simulink model "prueba"  (R2025b)
settings: Solver=VariableStepAuto  StartTime=0.0  StopTime=10.0  RelTol=1e-3
values from neighbouring files (symbols this model uses):
  bcx = 1.0e6    (= 1000000)    [parametros.m]
  bcy = 10.0e6    (= 10000000)    [parametros.m]
  bh_eq = bhm + bhd/(ih^2)    (= 18.0165289256)    [parametros.m]
  bhb = 100e6    (= 100000000)    [parametros.m]
  bhEb = 2.2e9    (= 2200000000)    [parametros.m]
  bhwu = 150    [parametros.m]
  bt = 90.0    (= 90)    [parametros.m]
  bt_eq = btm + btd/(it^2)    (= 6.002)    [parametros.m]
  btb = 5.0e6    (= 5000000)    [parametros.m]
  btw = 3.0e3    (= 3000)    [parametros.m]
  g = 9.80665    [parametros.m]
  Hc = 2.59    [parametros.m]
  ih = 22.0    (= 22)    [parametros.m]
  it = 30.0    (= 30)    [parametros.m]
  Jh_eq = J_hm_hb + J_hd_hEb/(ih^2)    (= 37.8512396694)    [parametros.m]
  Jt_eq = Jtm_tb + Jtd/(it^2)    (= 8.33333333333)    [parametros.m]
  Kcy = 1.8e9    (= 1800000000)    [parametros.m]
  khwu = 236e6    (= 236000000)    [parametros.m]
  Ki_h = (wn_h^2)*Jh_eq    (= 34.1607438017)    [parametros.m]
  Ki_t = (wn_t^2*Mt)/Kf    (= 320)    [parametros.m]
  Kp_h = 2*zitta_h*wn_h*Jh_eq    (= 79.1090909091)    [parametros.m]
  Kp_t = (2*zitta_t*wn_t*Mt)/Kf    (= 1120)    [parametros.m]
  Ktw = 480e3    (= 480000)    [parametros.m]
  Lh0 = 110    [parametros.m]
  lh_0 = Yt0 - yh_0    (= 25)    [parametros.m]
  Mc_max = 50000    [parametros.m]
  Ms = 15000    [parametros.m]
  Mt = 30000    [parametros.m]
  rhd = 0.75    [parametros.m]
  rtd = 0.50    (= 0.5)    [parametros.m]
  tau_hm = 1.0e-3    (= 0.001)    [parametros.m]
  tau_tm = 1.0e-3    (= 0.001)    [parametros.m]
  Thb_Max = 50e3    (= 50000)    [parametros.m]
  ThEb_Max = 1.1e6    (= 1100000)    [parametros.m]
  Thm_0 = Ms*g*rhd/(2*ih)    (= 2507.38210227)    [parametros.m]
  Thm_Max = 20e3    (= 20000)    [parametros.m]
  titahm_0 = yh_0/(rhd/(2*ih))    (= 1173.33333333)    [parametros.m]
  titatm_0 = xtd_0/(rtd/it)    (= 1500)    [parametros.m]
  Ts2 = 1e-3    (= 0.001)    [parametros.m]
  Ttb_Max = 5.0e3    (= 5000)    [parametros.m]
  Ttm_0 = 0    [parametros.m]
  Ttm_Max = 4.0e3    (= 4000)    [parametros.m]
  vlx_0 = 0    [parametros.m]
  vly_0 = 0    [parametros.m]
  vt_0 = 0    [parametros.m]
  whm_0 = 0    [parametros.m]
  whm_rated = vh_nom*2*ih/rhd    (= 88)    [parametros.m]
  wtm_0 = 0    [parametros.m]
  xl_0 = xt_0    (= 25)    [parametros.m]
  xt_0 = 25    [parametros.m]
  xtd_0 = xt_0    (= 25)    [parametros.m]
  yl_0 = Yt0 - l_0    (= 19.975067839)    [parametros.m]
  Yt0 = 45.0    (= 45)    [parametros.m]
undefined symbols (not defined in the file or in its folder): DiscIntNeverNeededParam, magnitude
libraries: simulink x1
settings Model: Creator=lauta  LastModifiedBy=lauta

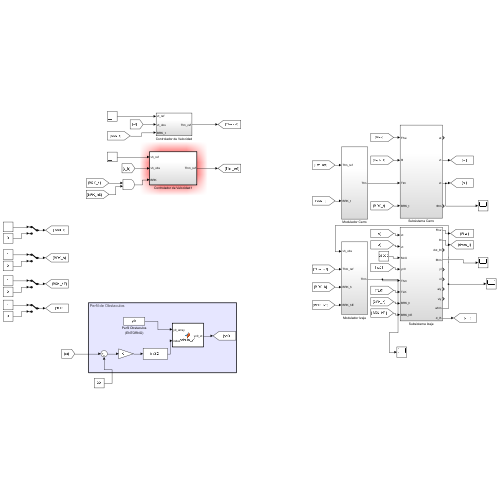
[thumbnail: Simulink's stored preview of the top-level diagram]
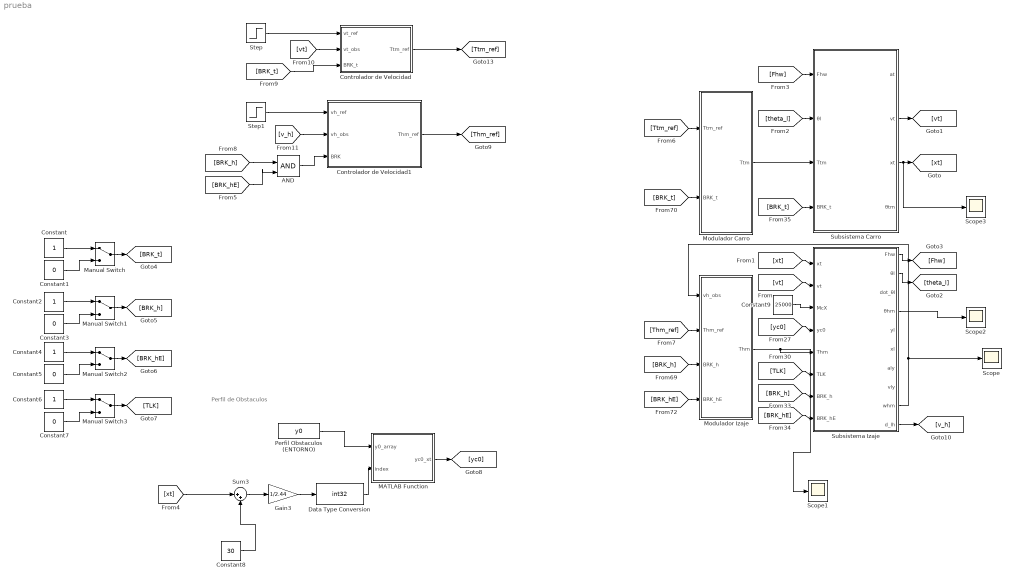
== system prueba ==
  note: Perfil de Obstaculos
  AND : Logic  IconShape=distinctive  AllPortsSameDT=off  OutDataTypeStr=boolean
  Constant{,2,4,6} (4 alike) : Constant
  Constant{1,3,5,7} (4 alike) : Constant  Value=0
  Constant8 : Constant  Value=30
  Constant9 : Constant  Value=25000
  Controlador de Velocidad : Subsystem
  Controlador de Velocidad1 : Subsystem  TreatAsAtomicUnit=on  SystemSampleTime=Ts2
  Data Type Conversion : DataTypeConversion  OutDataTypeStr=int32  RndMeth=Ceiling  SaturateOnIntegerOverflow=off
  Gain3 : Gain  Gain=1/2.44
  MATLAB Function : MATLAB Function  TreatAsAtomicUnit=on
  Manual Switch{,1..3} (4 alike) : ManualSwitch
  Modulador Carro : Subsystem
  Modulador Izaje : Subsystem
  Perfil Obstaculos (ENTORNO) : FromWorkspace  VariableName=y0
  Scope{,1..3} (4 alike) : Scope
      Scope settings: ActiveDisplayYMinimum=-16.360074628289411  ActiveDisplayYMaximum=147.24067165460474
      Scope1 settings: ActiveDisplayYMinimum=-1  ActiveDisplayYMaximum=1
      Scope2 settings: ActiveDisplayYMinimum=-1  ActiveDisplayYMaximum=1  DataLoggingVariableName=ScopeData2
      Scope3 settings: ActiveDisplayYMinimum=24.75610602663804  ActiveDisplayYMaximum=27.195045760257642  DataLoggingVariableName=ScopeData4
  Step : Step  SampleTime=0
  Step1 : Step  SampleTime=0
  Subsistema Carro : Subsystem
  Subsistema Izaje : Subsystem
  Sum3 : Sum  Inputs=|++
  wires:
  Subsistema Izaje/1(Fhw) -> [Fhw]
  Subsistema Izaje/9(whm) -> Scope/1, Modulador Izaje/1(vh_obs)
  [vt] -> Subsistema Izaje/2(vt)
  [BRK_t] -> Subsistema Carro/4(BRK_t)
  [xt] -> Subsistema Izaje/1(xt)
  Constant9/1 -> Subsistema Izaje/3(McX)
  Modulador Izaje/1(Thm) -> Scope1/1, Subsistema Izaje/5(Thm)
  [BRK_h] -> Subsistema Izaje/7(BRK_h)
  Subsistema Izaje/2(θl) -> [theta_l]
  Subsistema Carro/2(vt) -> [vt]
  [Fhw] -> Subsistema Carro/1(Fhw)
  [BRK_hE] -> Subsistema Izaje/8(BRK_hE)
  [theta_l] -> Subsistema Carro/2(θl)
  [BRK_h] -> Modulador Izaje/3(BRK_h)
  [yc0] -> Subsistema Izaje/4(yc0)
  [BRK_t] -> Modulador Carro/2(BRK_t)
  Subsistema Carro/3(xt) -> Scope3/1, [xt]
  [BRK_hE] -> Modulador Izaje/4(BRK_hE)
  Modulador Carro/1(Ttm) -> Subsistema Carro/3(Ttm)
  [TLK] -> Subsistema Izaje/6(TLK)
  Manual Switch/1 -> [BRK_t]
  Constant/1 -> Manual Switch/1
  Constant1/1 -> Manual Switch/2
  Constant3/1 -> Manual Switch1/2
  Constant2/1 -> Manual Switch1/1
  Manual Switch1/1 -> [BRK_h]
  Manual Switch2/1 -> [BRK_hE]
  Constant4/1 -> Manual Switch2/1
  Constant5/1 -> Manual Switch2/2
  Constant7/1 -> Manual Switch3/2
  Constant6/1 -> Manual Switch3/1
  Manual Switch3/1 -> [TLK]
  Gain3/1 -> Data Type Conversion/1
  Sum3/1 -> Gain3/1
  Perfil Obstaculos (ENTORNO)/1 -> MATLAB Function/1(y0_array)
  Data Type Conversion/1 -> MATLAB Function/2(index)
  [xt] -> Sum3/1
  Constant8/1 -> Sum3/2
  MATLAB Function/1(yc0_xt) -> [yc0]
  Subsistema Izaje/4(θhm) -> Scope2/1
  [Ttm_ref] -> Modulador Carro/1(Ttm_ref)
  [Thm_ref] -> Modulador Izaje/2(Thm_ref)
  Controlador de Velocidad/1(Ttm_ref) -> [Ttm_ref]
  Controlador de Velocidad1/1(Thm_ref) -> [Thm_ref]
  AND/1 -> Controlador de Velocidad1/3(BRK)
  [BRK_t] -> Controlador de Velocidad/3(BRK_t)
  [BRK_h] -> AND/1
  [BRK_hE] -> AND/2
  Step/1 -> Controlador de Velocidad/1(vt_ref)
  Step1/1 -> Controlador de Velocidad1/1(vh_ref)
  [vt] -> Controlador de Velocidad/2(vt_obs)
  Subsistema Izaje/10(d_lh) -> [v_h]
  [v_h] -> Controlador de Velocidad1/2(vh_obs)

== system prueba/Controlador de Velocidad ==
  vt_ref : Inport
  vt_obs : Inport  Port=2
  BRK_t : Inport  Port=3
  Discrete-Time Integrator : DiscreteIntegrator  IntegratorMethod=Integration: Trapezoidal  ExternalReset=level  SampleTime=-1  ICPrevOutput=DiscIntNeverNeededParam  ICPrevScaledInput=DiscIntNeverNeededParam
  Gain5 : Gain  Gain=Ki_t
  Gain6 : Gain  Gain=Kp_t
  NOT : Logic  Operator=NOT  IconShape=distinctive  AllPortsSameDT=off  OutDataTypeStr=boolean
  Sum6 : Sum  Inputs=+-
  Sum7 : Sum  Inputs=++|
  Ttm_ref : Outport
  wires:
  Sum6/1 -> Gain6/1, Discrete-Time Integrator/1  "e_v"
  Sum7/1 -> Ttm_ref/1
  Gain5/1 -> Sum7/2
  vt_ref/1 -> Sum6/1
  Gain6/1 -> Sum7/1
  vt_obs/1 -> Sum6/2
  Discrete-Time Integrator/1 -> Gain5/1
  BRK_t/1 -> NOT/1
  NOT/1 -> Discrete-Time Integrator/2

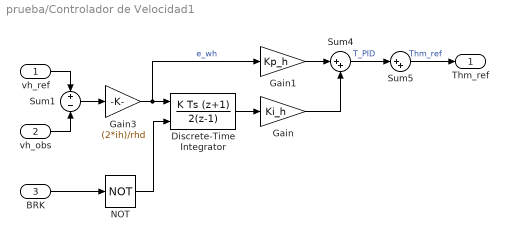
== system prueba/Controlador de Velocidad1 ==
  vh_ref : Inport
  vh_obs : Inport  Port=2
  BRK : Inport  Port=3
  Discrete-Time Integrator : DiscreteIntegrator  IntegratorMethod=Integration: Trapezoidal  ExternalReset=level  SampleTime=-1  ICPrevOutput=DiscIntNeverNeededParam  ICPrevScaledInput=DiscIntNeverNeededParam
  Gain : Gain  Gain=Ki_h
  Gain1 : Gain  Gain=Kp_h
  Gain3 : Gain  Gain=(2*ih)/rhd
  NOT : Logic  Operator=NOT  IconShape=distinctive  AllPortsSameDT=off  OutDataTypeStr=boolean
  Sum1 : Sum  Inputs=+-
  Sum4 : Sum  Inputs=|++
  Sum5 : Sum  Inputs=|++
  Thm_ref : Outport
  wires:
  Gain1/1 -> Sum4/1
  Sum1/1 -> Gain3/1
  vh_obs/1 -> Sum1/2
  Sum5/1 -> Thm_ref/1  "Thm_ref"
  Sum4/1 -> Sum5/1  "T_PID"
  vh_ref/1 -> Sum1/1
  Discrete-Time Integrator/1 -> Gain/1
  Gain/1 -> Sum4/2
  NOT/1 -> Discrete-Time Integrator/2
  BRK/1 -> NOT/1
  Gain3/1 -> Discrete-Time Integrator/1, Gain1/1  "e_wh"

== system prueba/Modulador Carro ==
  Ttm_ref : Inport
  BRK_t : Inport  Port=2
  Constant1 : Constant  Value=0
  Gain2 : Gain  Gain=1/tau_tm
  Integrator : Integrator  InitialCondition=Ttm_0
  Saturation : Saturate  UpperLimit=Ttm_Max  LowerLimit=-Ttm_Max
  Sum : Sum  Inputs=|+-
  Switch : Switch  Criteria=u2 > Threshold  SaturateOnIntegerOverflow=off  InputSameDT=off
  Ttm : Outport
  wires:
  Saturation/1 -> Sum/1  "Ttm_lim"
  Sum/1 -> Gain2/1
  Gain2/1 -> Integrator/1
  Integrator/1 -> Ttm/1, Sum/2
  Ttm_ref/1 -> Switch/1
  BRK_t/1 -> Switch/2
  Switch/1 -> Saturation/1
  Constant1/1 -> Switch/3

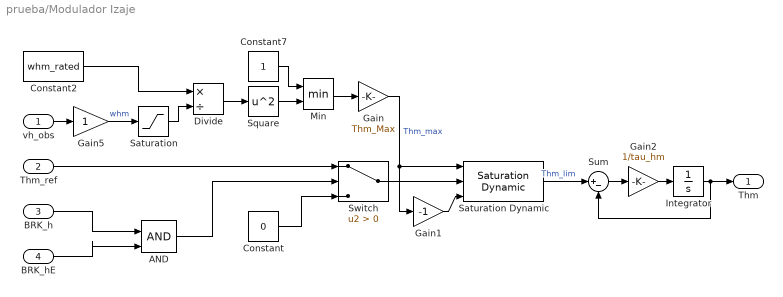
== system prueba/Modulador Izaje ==
  vh_obs : Inport
  Thm_ref : Inport  Port=2
  BRK_h : Inport  Port=3
  BRK_hE : Inport  Port=4
  AND : Logic  IconShape=distinctive  AllPortsSameDT=off  OutDataTypeStr=boolean
  Constant : Constant  Value=0
  Constant2 : Constant  Value=whm_rated
  Constant7 : Constant
  Divide : Product  Inputs=*/
  Gain : Gain  Gain=Thm_Max
  Gain1 : Gain  Gain=-1
  Gain2 : Gain  Gain=1/tau_hm
  Gain5 : Gain
  Integrator : Integrator  InitialCondition=Thm_0
  Min : MinMax  Inputs=2
  Saturation : Saturate  UpperLimit=inf  LowerLimit=whm_rated
  Saturation Dynamic : simulink/Discontinuities/Saturation Dynamic  OutMin=[]  OutMax=[]  OutDataTypeStr=Inherit: Same as second input  OutDataType=fixdt(1, 16)  OutScaling=2^-10  DoSatur=off
  Square : Math  Operator=square
  Sum : Sum  Inputs=|+-
  Switch : Switch  Criteria=u2 > Threshold  SaturateOnIntegerOverflow=off  InputSameDT=off
  Thm : Outport
  wires:
  Constant2/1 -> Divide/1
  Min/1 -> Gain/1
  Constant7/1 -> Min/1
  Gain/1 -> Gain1/1, Saturation Dynamic/1  "Thm_max"
  Saturation/1 -> Divide/2
  Square/1 -> Min/2
  Divide/1 -> Square/1
  vh_obs/1 -> Gain5/1
  Gain1/1 -> Saturation Dynamic/3
  Saturation Dynamic/1 -> Sum/1  "Thm_lim"
  Sum/1 -> Gain2/1
  Gain2/1 -> Integrator/1
  Integrator/1 -> Thm/1, Sum/2
  Thm_ref/1 -> Switch/1
  BRK_h/1 -> AND/1
  Switch/1 -> Saturation Dynamic/2
  BRK_hE/1 -> AND/2
  AND/1 -> Switch/2
  Gain5/1 -> Saturation/1  "whm"
  Constant/1 -> Switch/3

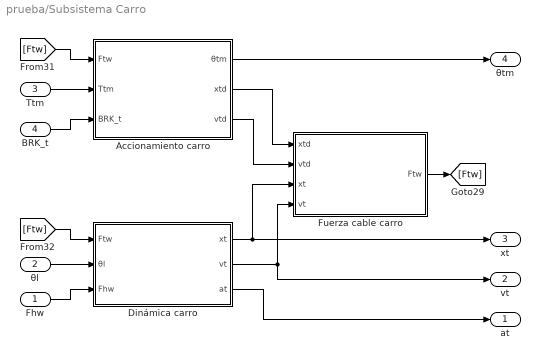
== system prueba/Subsistema Carro ==
  Fhw : Inport
  θl : Inport  Port=2
  Ttm : Inport  Port=3
  BRK_t : Inport  Port=4
  Accionamiento carro : Subsystem
  Dinámica carro : Subsystem
  Fuerza cable carro : Subsystem
  at : Outport
  vt : Outport  Port=2
  xt : Outport  Port=3
  θtm : Outport  Port=4
  wires:
  [Ftw] -> Accionamiento carro/1(Ftw)
  Accionamiento carro/1(θtm) -> θtm/1
  Dinámica carro/1(xt) -> Fuerza cable carro/3(xt), xt/1
  BRK_t/1 -> Accionamiento carro/3(BRK_t)
  [Ftw] -> Dinámica carro/1(Ftw)
  θl/1 -> Dinámica carro/2(θl)
  Ttm/1 -> Accionamiento carro/2(Ttm)
  Fuerza cable carro/1(Ftw) -> [Ftw]
  Dinámica carro/2(vt) -> Fuerza cable carro/4(vt), vt/1
  Accionamiento carro/2(xtd) -> Fuerza cable carro/1(xtd)
  Accionamiento carro/3(vtd) -> Fuerza cable carro/2(vtd)
  Fhw/1 -> Dinámica carro/3(Fhw)
  Dinámica carro/3(at) -> at/1

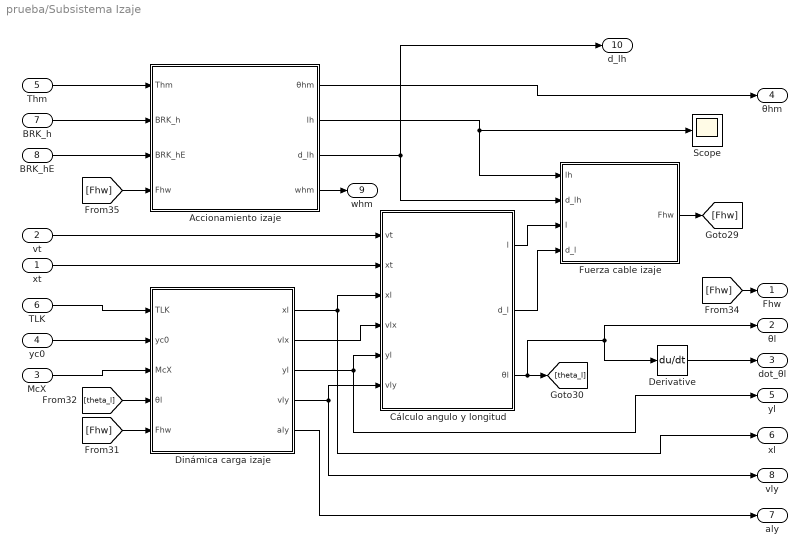
== system prueba/Subsistema Izaje ==
  xt : Inport
  vt : Inport  Port=2
  McX : Inport  Port=3
  yc0 : Inport  Port=4
  Thm : Inport  Port=5
  TLK : Inport  Port=6
  BRK_h : Inport  Port=7
  BRK_hE : Inport  Port=8
  Accionamiento izaje : Subsystem
  Cálculo angulo y longitud : Subsystem
  Derivative : Derivative
  Dinámica carga izaje : Subsystem
  Fuerza cable izaje : Subsystem
  Scope : Scope
      settings: ActiveDisplayYMinimum=-1  ActiveDisplayYMaximum=1  DataLoggingVariableName=ScopeData3
  Fhw : Outport
  θl : Outport  Port=2
  dot_θl : Outport  Port=3
  θhm : Outport  Port=4
  yl : Outport  Port=5
  xl : Outport  Port=6
  aly : Outport  Port=7
  vly : Outport  Port=8
  whm : Outport  Port=9
  d_lh : Outport  Port=10
  wires:
  vt/1 -> Cálculo angulo y longitud/1(vt)
  Accionamiento izaje/2(lh) -> Scope/1, Fuerza cable izaje/1(lh)
  yc0/1 -> Dinámica carga izaje/2(yc0)
  McX/1 -> Dinámica carga izaje/3(McX)
  Dinámica carga izaje/4(vly) -> vly/1, Cálculo angulo y longitud/6(vly)
  [Fhw] -> Accionamiento izaje/4(Fhw)
  [theta_l] -> Dinámica carga izaje/4(θl)
  xt/1 -> Cálculo angulo y longitud/2(xt)
  BRK_h/1 -> Accionamiento izaje/2(BRK_h)
  Dinámica carga izaje/1(xl) -> Cálculo angulo y longitud/3(xl), xl/1
  Dinámica carga izaje/2(vlx) -> Cálculo angulo y longitud/4(vlx)
  Fuerza cable izaje/1(Fhw) -> [Fhw]
  Cálculo angulo y longitud/1(l) -> Fuerza cable izaje/3(l)
  Accionamiento izaje/1(θhm) -> θhm/1
  Cálculo angulo y longitud/3(θl) -> θl/1, Derivative/1, [theta_l]
  TLK/1 -> Dinámica carga izaje/1(TLK)
  [Fhw] -> Dinámica carga izaje/5(Fhw)
  BRK_hE/1 -> Accionamiento izaje/3(BRK_hE)
  Thm/1 -> Accionamiento izaje/1(Thm)
  Dinámica carga izaje/3(yl) -> Cálculo angulo y longitud/5(yl), yl/1
  Cálculo angulo y longitud/2(d_l) -> Fuerza cable izaje/4(d_l)
  Accionamiento izaje/3(d_lh) -> d_lh/1, Fuerza cable izaje/2(d_lh)
  Dinámica carga izaje/5(aly) -> aly/1
  [Fhw] -> Fhw/1
  Derivative/1 -> dot_θl/1
  Accionamiento izaje/4(whm) -> whm/1

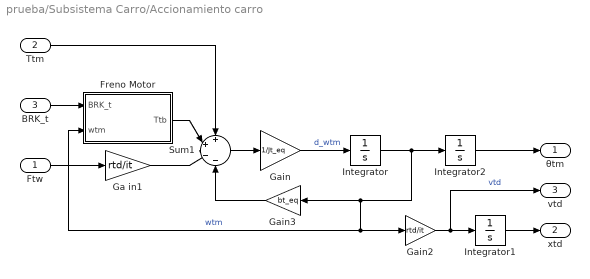
== system prueba/Subsistema Carro/Accionamiento carro ==
  Ftw : Inport
  Ttm : Inport  Port=2
  BRK_t : Inport  Port=3
  Freno Motor : Subsystem
  Ga in1 : Gain  Gain=rtd/it
  Gain : Gain  Gain=1/Jt_eq
  Gain2 : Gain  Gain=rtd/it
  Gain3 : Gain  Gain=bt_eq
  Integrator : Integrator  InitialCondition=wtm_0
  Integrator1 : Integrator  InitialCondition=xtd_0
  Integrator2 : Integrator  InitialCondition=titatm_0
  Sum1 : Sum  Inputs=++--
  θtm : Outport
  xtd : Outport  Port=2
  vtd : Outport  Port=3
  wires:
  Sum1/1 -> Gain/1
  Integrator/1 -> Gain2/1, Freno Motor/2(wtm), Gain3/1, Integrator2/1  "wtm"
  Gain2/1 -> Integrator1/1, vtd/1  "vtd"
  Ttm/1 -> Sum1/1
  Gain/1 -> Integrator/1  "d_wtm"
  BRK_t/1 -> Freno Motor/1(BRK_t)
  Integrator1/1 -> xtd/1
  Ftw/1 -> Ga in1/1
  Ga in1/1 -> Sum1/3
  Freno Motor/1(Ttb) -> Sum1/2
  Gain3/1 -> Sum1/4
  Integrator2/1 -> θtm/1

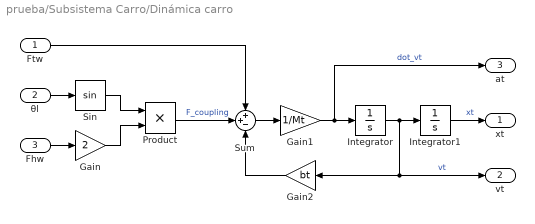
== system prueba/Subsistema Carro/Dinámica carro ==
  Ftw : Inport
  θl : Inport  Port=2
  Fhw : Inport  Port=3
  Gain : Gain  Gain=2
  Gain1 : Gain  Gain=1/Mt
  Gain2 : Gain  Gain=bt
  Integrator : Integrator  InitialCondition=vt_0
  Integrator1 : Integrator  InitialCondition=xt_0
  Product : Product
  Sin : Trigonometry
  Sum : Sum  Inputs=++-
  xt : Outport
  vt : Outport  Port=2
  at : Outport  Port=3
  wires:
  Gain1/1 -> at/1, Integrator/1  "dot_vt"
  Integrator/1 -> Gain2/1, vt/1, Integrator1/1  "vt"
  Gain2/1 -> Sum/3
  Sum/1 -> Gain1/1
  Integrator1/1 -> xt/1  "xt"
  Fhw/1 -> Gain/1
  Gain/1 -> Product/2
  θl/1 -> Sin/1
  Sin/1 -> Product/1
  Product/1 -> Sum/2  "F_coupling"
  Ftw/1 -> Sum/1

== system prueba/Subsistema Carro/Fuerza cable carro ==
  xtd : Inport
  vtd : Inport  Port=2
  xt : Inport  Port=3
  vt : Inport  Port=4
  Gain : Gain  Gain=Ktw
  Gain1 : Gain  Gain=btw
  Sum : Sum  Inputs=+-
  Sum1 : Sum
  Sum2 : Sum  Inputs=+-
  Ftw : Outport
  wires:
  xtd/1 -> Sum/1
  Gain1/1 -> Sum1/2
  Sum/1 -> Gain/1
  xt/1 -> Sum/2
  Sum2/1 -> Gain1/1
  Gain/1 -> Sum1/1
  vt/1 -> Sum2/2
  Sum1/1 -> Ftw/1  "Ftw"
  vtd/1 -> Sum2/1

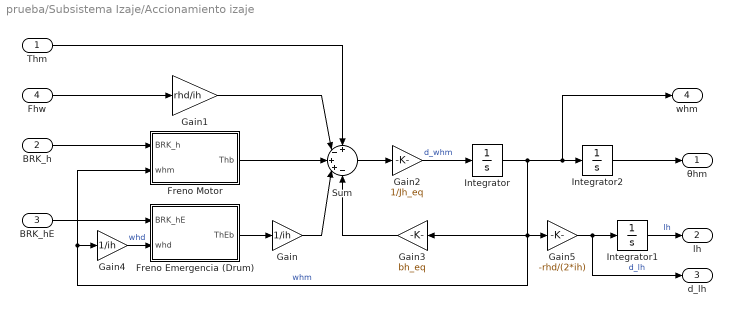
== system prueba/Subsistema Izaje/Accionamiento izaje ==
  Thm : Inport
  BRK_h : Inport  Port=2
  BRK_hE : Inport  Port=3
  Fhw : Inport  Port=4
  Freno Emergencia (Drum) : Subsystem
  Freno Motor : Subsystem
  Gain : Gain  Gain=1/ih
  Gain1 : Gain  Gain=rhd/ih
  Gain2 : Gain  Gain=1/Jh_eq
  Gain3 : Gain  Gain=bh_eq
  Gain4 : Gain  Gain=1/ih
  Gain5 : Gain  Gain=-rhd/(2*ih)
  Integrator : Integrator  InitialCondition=whm_0
  Integrator1 : Integrator  InitialCondition=lh_0
  Integrator2 : Integrator  InitialCondition=titahm_0
  Sum : Sum  Inputs=+-++-
  θhm : Outport
  lh : Outport  Port=2
  d_lh : Outport  Port=3
  whm : Outport  Port=4
  wires:
  Gain5/1 -> d_lh/1, Integrator1/1  "d_lh"
  Integrator/1 -> Gain3/1, Freno Motor/2(whm), Gain4/1, Gain5/1, whm/1, Integrator2/1  "whm"
  Freno Emergencia (Drum)/1(ThEb) -> Gain/1
  Gain3/1 -> Sum/5
  BRK_h/1 -> Freno Motor/1(BRK_h)
  Gain/1 -> Sum/4
  Gain2/1 -> Integrator/1  "d_whm"
  Sum/1 -> Gain2/1
  Gain4/1 -> Freno Emergencia (Drum)/2(whd)  "whd"
  BRK_hE/1 -> Freno Emergencia (Drum)/1(BRK_hE)
  Fhw/1 -> Gain1/1
  Freno Motor/1(Thb) -> Sum/3
  Gain1/1 -> Sum/2
  Integrator1/1 -> lh/1  "lh"
  Integrator2/1 -> θhm/1
  Thm/1 -> Sum/1

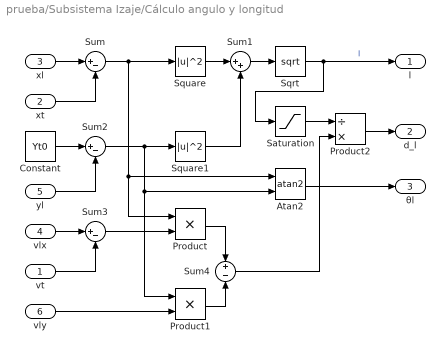
== system prueba/Subsistema Izaje/Cálculo angulo y longitud ==
  vt : Inport
  xt : Inport  Port=2
  xl : Inport  Port=3
  vlx : Inport  Port=4
  yl : Inport  Port=5
  vly : Inport  Port=6
  Atan2 : Trigonometry  Operator=atan2
  Constant : Constant  Value=Yt0
  Product : Product
  Product1 : Product
  Product2 : Product  Inputs=/*
  Saturation : Saturate  UpperLimit=inf  LowerLimit=0.1
  Sqrt : Sqrt
  Square : Math  Operator=magnitude^2
  Square1 : Math  Operator=magnitude^2
  Sum : Sum  Inputs=|+-
  Sum1 : Sum  Inputs=|++
  Sum2 : Sum  Inputs=|+-
  Sum3 : Sum  Inputs=|+-
  Sum4 : Sum  Inputs=+-
  l : Outport
  d_l : Outport  Port=2
  θl : Outport  Port=3
  wires:
  Product2/1 -> d_l/1
  Sqrt/1 -> l/1, Saturation/1  "l"
  Sum1/1 -> Sqrt/1
  Sum2/1 -> Product1/1, Atan2/2, Square1/1
  Sum/1 -> Product/1, Atan2/1, Square/1
  yl/1 -> Sum2/2
  Atan2/1 -> θl/1
  vly/1 -> Product1/2
  xl/1 -> Sum/1
  Constant/1 -> Sum2/1
  Sum3/1 -> Product/2
  Square1/1 -> Sum1/2
  vt/1 -> Sum3/2
  Sum4/1 -> Product2/2
  vlx/1 -> Sum3/1
  xt/1 -> Sum/2
  Square/1 -> Sum1/1
  Product1/1 -> Sum4/2
  Product/1 -> Sum4/1
  Saturation/1 -> Product2/1

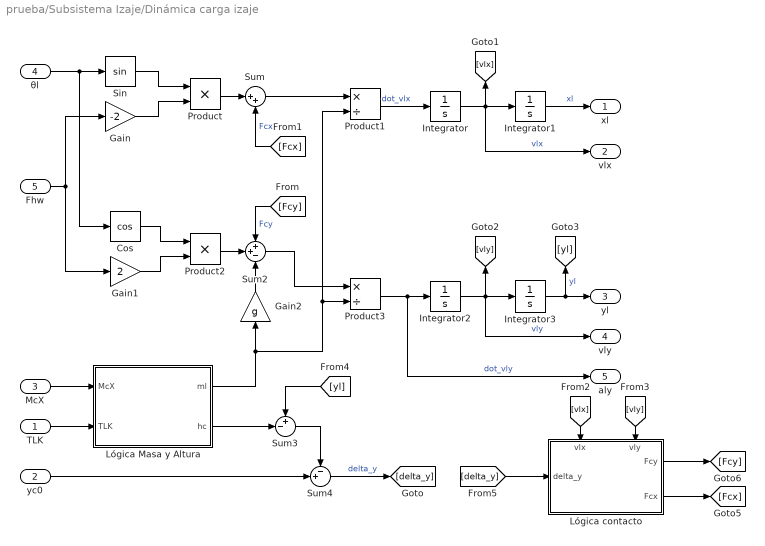
== system prueba/Subsistema Izaje/Dinámica carga izaje ==
  TLK : Inport
  yc0 : Inport  Port=2
  McX : Inport  Port=3
  θl : Inport  Port=4
  Fhw : Inport  Port=5
  Cos : Trigonometry  Operator=cos
  Gain : Gain  Gain=-2
  Gain1 : Gain  Gain=2
  Gain2 : Gain  Gain=g
  Integrator : Integrator  InitialCondition=vlx_0
  Integrator1 : Integrator  InitialCondition=xl_0
  Integrator2 : Integrator  InitialCondition=vly_0
  Integrator3 : Integrator  InitialCondition=yl_0
  Lógica Masa y Altura : Subsystem
  Lógica contacto : Subsystem
      settings: PortSchema="{\"entries\":[{\"content\":{\"sides\":[{\"content\":{\"connectorIds\":[\"In1\"]},\"type\":\"ConnectorPlacement.EquallySpacedRectSide\",\"uuid\":\"20a8b2c4-d5cf-44ce-93ec-929b996a0905\"},{\"content\":{\"connectorIds\":[\"Out1\",\"Out2\"],\"side\":\"RIGHT\"},\"type\":\"ConnectorPlacement.EquallySpacedRectSide\",\"uuid\":\"396e1f2e-cf71-48dc-8d57-a3e2695dfff1\"},{\"content\":{\"connectorIds\":[\"In2\",\"In3\"],\"side\":\"TOP\"},\"type\":\"ConnectorPlacement.EquallySpacedRectSide\",\"uuid\":\"e66c0478-9682-41e1-9b77-d2d789a9c323\"}]},\"type\":\"ConnectorPlacement.EquallySpacedConnector\",\"uuid\":\"193dabd2-f524-433a-b6ef-c1cab585578e\"}],\"packageUris\":[\"http://schema.mathworks.com/mf0/Connector/R2020b\"],\"version\":\"1.0\"}"
  Product : Product
  Product1 : Product  Inputs=*/
  Product2 : Product
  Product3 : Product  Inputs=*/
  Sin : Trigonometry
  Sum : Sum  Inputs=|++
  Sum2 : Sum  Inputs=++-
  Sum3 : Sum  Inputs=+-|
  Sum4 : Sum  Inputs=-+|
  xl : Outport
  vlx : Outport  Port=2
  yl : Outport  Port=3
  vly : Outport  Port=4
  aly : Outport  Port=5
  wires:
  θl/1 -> Sin/1, Cos/1
  Integrator/1 -> vlx/1, Integrator1/1, [vlx]  "vlx"
  Sum3/1 -> Sum4/1
  Sin/1 -> Product/1
  Gain/1 -> Product/2
  [Fcy] -> Sum2/1  "Fcy"
  Integrator2/1 -> vly/1, Integrator3/1, [vly]  "vly"
  Integrator3/1 -> yl/1, [yl]  "yl"
  Fhw/1 -> Gain1/1, Gain/1
  [Fcx] -> Sum/2  "Fcx"
  Product/1 -> Sum/1
  Product1/1 -> Integrator/1  "dot_vlx"
  Gain2/1 -> Sum2/3
  Cos/1 -> Product2/1
  Gain1/1 -> Product2/2
  [yl] -> Sum3/1
  Product2/1 -> Sum2/2
  yc0/1 -> Sum4/2
  Sum2/1 -> Product3/1
  Product3/1 -> aly/1, Integrator2/1  "dot_vly"
  Sum/1 -> Product1/1
  Integrator1/1 -> xl/1  "xl"
  Sum4/1 -> [delta_y]  "delta_y"
  Lógica contacto/1(Fcy) -> [Fcy]
  Lógica contacto/2(Fcx) -> [Fcx]
  Lógica Masa y Altura/1(ml) -> Product1/2, Product3/2, Gain2/1
  McX/1 -> Lógica Masa y Altura/1(McX)
  TLK/1 -> Lógica Masa y Altura/2(TLK)
  Lógica Masa y Altura/2(hc) -> Sum3/2
  [vlx] -> Lógica contacto/2(vlx)
  [vly] -> Lógica contacto/3(vly)
  [delta_y] -> Lógica contacto/1(delta_y)

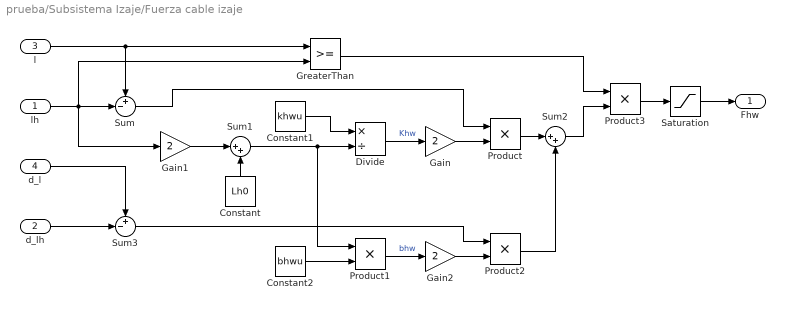
== system prueba/Subsistema Izaje/Fuerza cable izaje ==
  lh : Inport
  d_lh : Inport  Port=2
  l : Inport  Port=3
  d_l : Inport  Port=4
  Constant : Constant  Value=Lh0
  Constant1 : Constant  Value=khwu
  Constant2 : Constant  Value=bhwu
  Divide : Product  Inputs=*/  RndMeth=Zero  SaturateOnIntegerOverflow=on
  Gain : Gain  Gain=2
  Gain1 : Gain  Gain=2
  Gain2 : Gain  Gain=2
  GreaterThan : RelationalOperator  OutDataTypeStr=boolean  RndMeth=Simplest  InputSameDT=off
  Product{,1..3} (4 alike) : Product
  Saturation : Saturate  UpperLimit=inf  LowerLimit=0
  Sum : Sum  Inputs=+-|
  Sum1 : Sum  Inputs=|++
  Sum2 : Sum  Inputs=|++
  Sum3 : Sum  Inputs=+-|
  Fhw : Outport
  wires:
  Constant/1 -> Sum1/2
  Constant2/1 -> Product1/2
  Sum1/1 -> Divide/2, Product1/1
  lh/1 -> Sum/2, GreaterThan/2, Gain1/1
  Product/1 -> Sum2/1
  Gain1/1 -> Sum1/1
  l/1 -> Sum/1, GreaterThan/1
  Product2/1 -> Sum2/2
  Product3/1 -> Saturation/1
  GreaterThan/1 -> Product3/1
  d_lh/1 -> Sum3/2
  Constant1/1 -> Divide/1
  Product1/1 -> Gain2/1  "bhw"
  Sum/1 -> Product/1
  Gain2/1 -> Product2/2
  Divide/1 -> Gain/1  "Khw"
  Sum2/1 -> Product3/2
  Sum3/1 -> Product2/1
  d_l/1 -> Sum3/1
  Gain/1 -> Product/2
  Saturation/1 -> Fhw/1

== system prueba/Subsistema Carro/Accionamiento carro/Freno Motor ==
  BRK_t : Inport
  wtm : Inport  Port=2
  Constant : Constant  Value=0
  Gain3 : Gain  Gain=-Ttb_Max
  Gain4 : Gain  Gain=btb
  Switch : Switch  Criteria=u2 > Threshold  SaturateOnIntegerOverflow=off  InputSameDT=off
  Tanh : Trigonometry  Operator=tanh
  Ttb : Outport
  wires:
  BRK_t/1 -> Switch/2
  Constant/1 -> Switch/1
  wtm/1 -> Gain4/1
  Gain4/1 -> Tanh/1
  Tanh/1 -> Gain3/1
  Gain3/1 -> Switch/3
  Switch/1 -> Ttb/1

== system prueba/Subsistema Izaje/Accionamiento izaje/Freno Emergencia (Drum) ==
  BRK_hE : Inport
  whd : Inport  Port=2
  Constant : Constant  Value=0
  Gain3 : Gain  Gain=-ThEb_Max
  Gain4 : Gain  Gain=bhEb
  Switch : Switch  Criteria=u2 > Threshold  SaturateOnIntegerOverflow=off  InputSameDT=off
  Tanh : Trigonometry  Operator=tanh
  ThEb : Outport
  wires:
  BRK_hE/1 -> Switch/2
  Gain3/1 -> Switch/3
  Constant/1 -> Switch/1
  whd/1 -> Gain4/1
  Gain4/1 -> Tanh/1
  Tanh/1 -> Gain3/1
  Switch/1 -> ThEb/1

== system prueba/Subsistema Izaje/Accionamiento izaje/Freno Motor ==
  BRK_h : Inport
  whm : Inport  Port=2
  Constant : Constant  Value=0
  Gain3 : Gain  Gain=-Thb_Max
  Gain4 : Gain  Gain=bhb
  Switch : Switch  Criteria=u2 > Threshold  SaturateOnIntegerOverflow=off  InputSameDT=off
  Tanh : Trigonometry  Operator=tanh
  Thb : Outport
  wires:
  BRK_h/1 -> Switch/2
  Gain3/1 -> Switch/3
  Constant/1 -> Switch/1
  whm/1 -> Gain4/1
  Gain4/1 -> Tanh/1
  Tanh/1 -> Gain3/1
  Switch/1 -> Thb/1

== system prueba/Subsistema Izaje/Dinámica carga izaje/Lógica Masa y Altura ==
  McX : Inport
  TLK : Inport  Port=2
  Constant : Constant  Value=Ms
  Constant1 : Constant  Value=0
  Constant2 : Constant  Value=Hc
  Rate Limiter : RateLimiter  Commented=through  RisingSlewLimit=Mc_max/0.1  FallingSlewLimit=-Mc_max/0.1  SampleTimeMode=inherited  InitialCondition=Ms
  Sum1 : Sum  Inputs=|++
  Switch : Switch  Criteria=u2 > Threshold  SaturateOnIntegerOverflow=off  InputSameDT=off
  Switch1 : Switch  Criteria=u2 > Threshold  SaturateOnIntegerOverflow=off  InputSameDT=off
  ml : Outport
  hc : Outport  Port=2
  wires:
  Sum1/1 -> Switch/1
  Constant2/1 -> Switch1/1
  TLK/1 -> Switch1/2, Switch/2
  Constant/1 -> Switch/3, Sum1/2
  Constant1/1 -> Switch1/3
  McX/1 -> Sum1/1
  Switch/1 -> Rate Limiter/1
  Rate Limiter/1 -> ml/1
  Switch1/1 -> hc/1

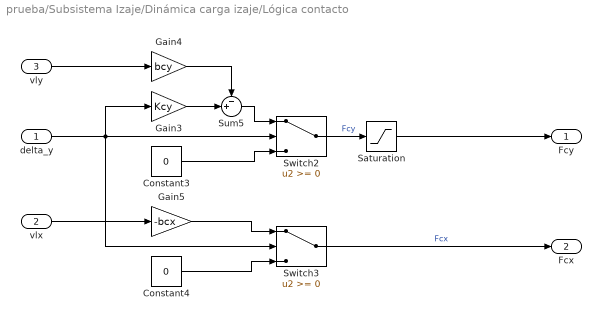
== system prueba/Subsistema Izaje/Dinámica carga izaje/Lógica contacto ==
  delta_y : Inport
  vlx : Inport  Port=2
  vly : Inport  Port=3
  Constant3 : Constant  Value=0
  Constant4 : Constant  Value=0
  Gain3 : Gain  Gain=Kcy
  Gain4 : Gain  Gain=bcy
  Gain5 : Gain  Gain=-bcx
  Saturation : Saturate  UpperLimit=60e5  LowerLimit=0
  Sum5 : Sum  Inputs=-+|
  Switch2 : Switch  SaturateOnIntegerOverflow=off  InputSameDT=off
  Switch3 : Switch  SaturateOnIntegerOverflow=off  InputSameDT=off
  Fcy : Outport
  Fcx : Outport  Port=2
  wires:
  Sum5/1 -> Switch2/1
  vlx/1 -> Gain5/1
  Gain4/1 -> Sum5/1
  vly/1 -> Gain4/1
  Constant4/1 -> Switch3/3
  Gain5/1 -> Switch3/1
  Gain3/1 -> Sum5/2
  delta_y/1 -> Switch3/2, Gain3/1, Switch2/2
  Constant3/1 -> Switch2/3
  Switch2/1 -> Saturation/1  "Fcy"
  Switch3/1 -> Fcx/1  "Fcx"
  Saturation/1 -> Fcy/1

== matlab function prueba/MATLAB Function ==
  data: y0_array input; yc0_xt output; index input
function yc0_xt= calcula_y0(y0_array,index)
yc0_xt = y0_array(index);
